simulink model "Spider_4leg_rotate_Ver0"  (R2024a)
settings: Solver=ode4  StartTime=0.0  StopTime=path_duration  FixedStep=0.01  RelTol=1e-3
PostLoadFcn:
  | addpath(fileparts(get_param('Spider_4leg_rotate_Ver0','FileName')));
InitFcn:
  | % Record inline model settings for the viewer; algorithms do not read this struct.
  | v0Model = 'Spider_4leg_rotate_Ver0';
  | v0Rt = sfroot;
  | v0W = v0Rt.find('-isa','Stateflow.EMChart','Path',[v0Model '/WPG']);
  | v0I = v0Rt.find('-isa','Stateflow.EMChart','Path',[v0Model '/IK_spider']);
  | v0F = v0Rt.find('-isa','Stateflow.EMChart','Path',[v0Model '/FK_spider']);
  | v0C = v0Rt.find('-isa','Stateflow.EMChart','Path',[v0Model '/COM_spider']);
  | v0Read = @(s,n) str2double(regexp(s,['(?m)^\s*' n '\s*=\s*([-+0-9.eE]+)\s*;'],'tokens','once'));
  | % Parse only numeric vector literals; no code is evaluated.
  | v0Literal = regexp(v0W.Script,'(?m)^\s*phi_leg\s*=\s*\[([0-9.,\s]+)\]','tokens','once');
  | v0Phase = sscanf(strrep(v0Literal{1},',',' '),'%f')';
  | v0Literal = regexp(v0C.Script,'(?m)^\s*com_offset\s*=\s*\[([-+0-9.eE,\s]+)\]','tokens','once');
  | v0Offset = sscanf(strrep(v0Literal{1},',',' '),'%f')';
  | v0P = struct;
  | v0P.FORMAT_VERSION = 1;
  | v0P.L = [v0Read(v0I.Script,'l1'),v0Read(v0I.Script,'l2'),v0Read(v0I.Script,'l3')];
  | v0cd = v0Read(v0W.Script,'cd');
  | v0cr = v0Read(v0W.Script,'cr');
  | v0P.HIP = [v0cd/2 v0cr/2;v0cd/2 -v0cr/2;-v0cd/2 -v0cr/2;-v0cd/2 v0cr/2];
  | v0P.STANCE = [v0Read(v0W.Script,'dx0'),v0Read(v0W.Script,'dy0')];
  | v0Switch = get_param([v0Model '/Direction'],'sw');
  | assert(ismember(v0Switch,{'0','1'}),'Ver0: invalid turn switch.');
  | v0Direction = 2*str2double(v0Switch)-1;
  | v0Base = sscanf(regexprep(get_param([v0Model '/COM0'],'Value'),'[\[\],]',' '),'%f');
  | assert(numel(v0Base)==3,'Ver0: COM0 must be a numeric [X Y Z] vector.');
  | v0P.BODY_H = v0Base(3);
  | v0P.STEP = 0;
  | v0P.T = str2double(get_param([v0Model '/T'],'Value'));
  | v0P.V = 0;
  | v0P.LIFT = v0Read(v0W.Script,'h');
  | v0P.SHIFT_X = v0Read(v0W.Script,'L_shift');
  | v0P.SHIFT_Y = v0Read(v0W.Script,'W_shift');
  | v0P.PHI = v0Phase;
  | if v0Direction > 0
  |     v0P.PHI = v0Phase([2 1 4 3]);
  | end
  | v0P.PREP = v0Read(v0W.Script,'beta_prep');
  | v0P.SWING = v0Read(v0W.Script,'beta_swing');
  | v0P.TOUCH = v0Read(v0W.Script,'beta_touch');
  | v0P.HEADING_DEG = str2double(get_param([v0Model '/phi0'],'Value'));
  | v0P.DT = str2double(get_param(v0Model,'FixedStep'));
  | v0Angle = str2double(get_param([v0Model '/Angle'],'Value'));
  | v0N = str2double(get_param([v0Model '/N'],'Value'));
  | assert(isfinite(v0Angle) && v0Angle>0 && v0Angle<=90,'Ver0: Angle must be in (0,90] degrees.');
  | assert(isfinite(v0N) && v0N>=4 && v0N<=200 && v0N==floor(v0N),'Ver0: N must be an integer in [4,200].');
  | v0Period = v0N*v0P.T;
  | assignin(get_param(v0Model,'ModelWorkspace'),'path_duration',v0Period);
  | assignin(get_param(v0Model,'ModelWorkspace'),'path_record',[3 v0Angle*pi/180 0 v0Period v0Direction 1]);
  | v0Stop = get_param(v0Model,'StopTime');
  | if strcmp(v0Stop,'path_duration')
  |     v0StopValue = v0Period;
  | else
  |     v0StopValue = str2double(v0Stop);
  | end
  | assert(isfinite(v0StopValue) && v0StopValue>0,'Ver0: Stop Time must be path_duration or a positive number.');
  | v0P.N_CYCLES = (v0StopValue-str2double(get_param(v0Model,'StartTime')))/v0P.T;
  | v0P.MASS_BODY = v0Read(v0C.Script,'m0')/1000;
  | v0P.MASS_LINK = [v0Read(v0C.Script,'m1'),v0Read(v0C.Script,'m2'),v0Read(v0C.Script,'m3')]/1000;
  | v0P.COM_OFFSET = v0Offset;
  | v0P.MARGIN_GUIDE = 0.005;
  | v0P.JOINT_TRIM = [0 -7 6;0 1.5 -3;4 -8 8;-6 -6 5];
  | v0P.SERVO_LO = [20 30 30];
  | v0P.SERVO_HI = [165 150 150];
  | assert(v0cd==v0Read(v0F.Script,'cd') && v0cr==v0Read(v0F.Script,'cr'),'Ver0: body dimensions differ between WPG and FK.');
  | assert(isequal(v0P.L,[v0Read(v0F.Script,'l1'),v0Read(v0F.Script,'l2'),v0Read(v0F.Script,'l3')]),'Ver0: link lengths differ between IK and FK.');
  | assert(v0P.DT==v0Read(v0C.Script,'dt') && v0P.DT==str2double(get_param([v0Model '/Delay1'],'SampleTime')),'Ver0: time step differs between solver, COM and Delay1.');
  | assert(v0P.PREP==0.75 && isequal(v0P.PHI,[.75 .5 .25 0] + (v0Direction>0)*[-.25 .25 -.25 .25]) && v0P.PREP<v0P.SWING && v0P.SWING<v0P.TOUCH && v0P.TOUCH<1,'Ver0: invalid phase schedule.');
  | assert(isfinite(v0P.T) && v0P.T>0 && v0P.V==0 && v0P.DT>0 && all(isfinite(v0P.L)) && all(v0P.L>0),'Ver0: invalid numeric parameter.');
  | assignin(get_param(v0Model,'ModelWorkspace'),'P',v0P);
  | clear v0Model v0Rt v0W v0I v0F v0C v0Read v0Vector v0Literal v0Phase v0Offset v0P v0cd v0cr v0Base
  | v0Root = sfroot;
  | v0Ref = v0Root.find('-isa','Stateflow.EMChart','Path',['Spider_4leg_rotate_Ver0' '/COM_ref']);
  | v0Wpg = v0Root.find('-isa','Stateflow.EMChart','Path',['Spider_4leg_rotate_Ver0' '/WPG']);
  | v0A = extractAfter(string(v0Ref.Script),'function pose = path_pose');
  | v0B = extractAfter(string(v0Wpg.Script),'function pose = path_pose');
  | assert(v0A==v0B,'Ver0: path_pose differs between COM_ref and WPG.');
  | clear v0R v0U v0Length v0Type v0Period v0Stop v0StopValue v0Root v0Ref v0Wpg v0A v0B
  | 
  | clear v0Switch v0Direction
  | clear v0Angle v0N
model workspace (MAT data in the model file):
  P.FORMAT_VERSION = 1
  P.L = [0.039 0.072 0.108]
  P.HIP = [0.0465  0.0445; 0.0465  -0.0445; -0.0465  -0.0445; -0.0465  0.0445]
  P.STANCE = [0.053 0.053]
  P.BODY_H = 0.088
  P.STEP = 0
  P.T = 12
  P.V = 0
  P.LIFT = 0.03
  P.SHIFT_X = 0.008
  P.SHIFT_Y = 0.017
  P.PHI = [0.75 0.5 0.25 0]
  P.PREP = 0.75
  P.SWING = 0.8
  P.TOUCH = 0.92
  P.HEADING_DEG = 0
  P.DT = 0.01
  P.N_CYCLES = 10
  P.MASS_BODY = 0.2
  P.MASS_LINK = [0.0134 0.0134 0.0134]
  P.COM_OFFSET = [0 0 0]
  P.MARGIN_GUIDE = 0.005
  P.JOINT_TRIM = [0  -7  6; 0  1.5  -3; 4  -8  8; -6  -6  5]
  P.SERVO_LO = [20 30 30]
  P.SERVO_HI = [165 150 150]
  path_duration = 120
  path_record = [3 1.57079632679 0 120 1 1]
settings Model: Creator=Huan  LastModifiedBy=hamin
settings RTWCC: GPUComputeCapability=3.5

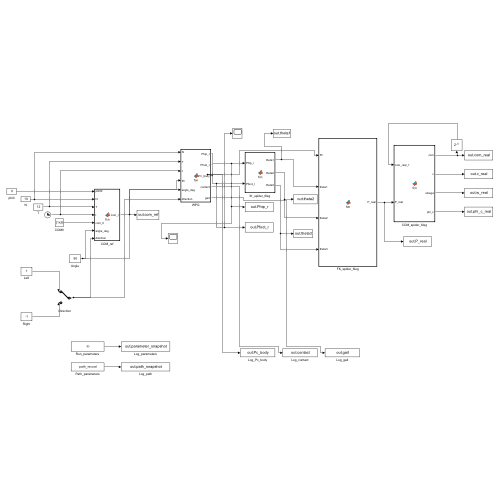
[thumbnail: Simulink's stored preview of the top-level diagram]
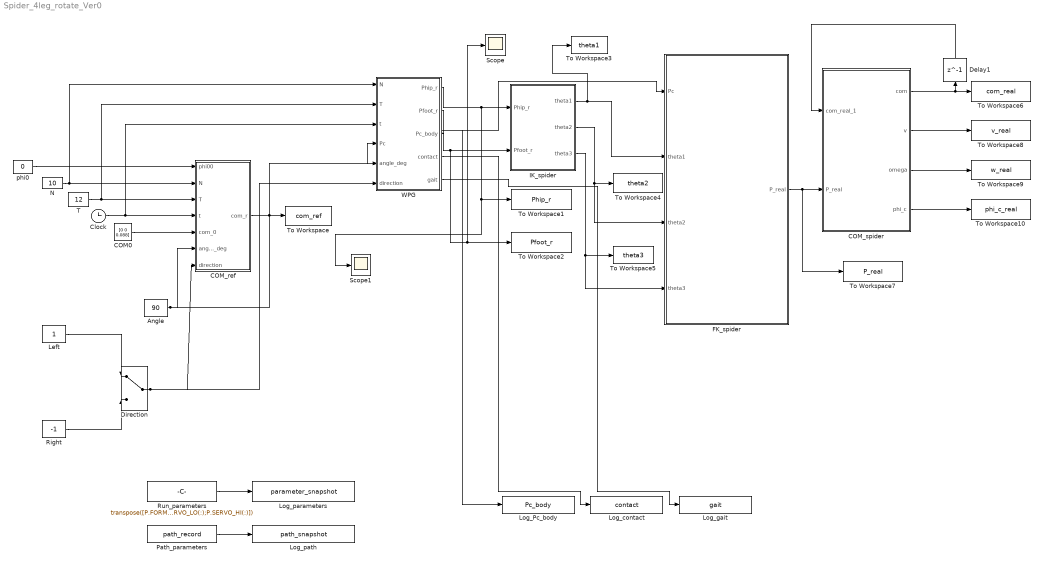
== system Spider_4leg_rotate_Ver0 ==
  Angle : Constant  Value=90
  COM0 : Constant  Value=[0 0 0.088]
  COM_ref : MATLAB Function  TreatAsAtomicUnit=on
  COM_spider : MATLAB Function  TreatAsAtomicUnit=on
  Clock : Clock
  Delay1 : Delay  DelayLength=1  InitialCondition=[0 0 -1 0]  SampleTime=0.01
  Direction : ManualSwitch
  FK_spider : MATLAB Function  TreatAsAtomicUnit=on
  IK_spider : MATLAB Function  TreatAsAtomicUnit=on
  Left : Constant
  Log_Pc_body : ToWorkspace  VariableName=Pc_body  SaveFormat=Timeseries  SampleTime=-1
  Log_contact : ToWorkspace  VariableName=contact  SaveFormat=Timeseries  SampleTime=-1
  Log_gait : ToWorkspace  VariableName=gait  SaveFormat=Timeseries  SampleTime=-1
  Log_parameters : ToWorkspace  VariableName=parameter_snapshot  SaveFormat=Timeseries  SampleTime=-1
      settings: MaxDataPoints=1
  Log_path : ToWorkspace  VariableName=path_snapshot  SaveFormat=Timeseries  SampleTime=-1
  N : Constant  Value=10
  Path_parameters : Constant  Value=path_record
  Right : Constant  Value=-1
  Run_parameters : Constant  Value=transpose([P.FORMAT_VERSION(:);P.L(:);P.HIP(:);P.STANCE(:);P.BODY_H(:);P.STEP(:);P.T(:);P.V(:);P.LIFT(:);P.SHIFT_X(:);P.SHIFT_Y(:);P.PHI(:);P.PREP(:);P.SWING(:);P.TOUCH(:);P.HEADING_DEG(:);P.DT(:);P.N_CYCLES(:);P.MASS_BODY(:);P.MASS_LINK(:);P.COM_OFFSET(:);P.MARGIN_GUIDE(:);P.JOINT_TRIM(:);P.SERVO_LO(:);P.SERVO_HI(:)])
  Scope : Scope
  Scope1 : Scope
  T : Constant  Value=12
  To Workspace : ToWorkspace  VariableName=com_ref  SaveFormat=Timeseries  SampleTime=-1
  To Workspace1 : ToWorkspace  VariableName=Phip_r  SaveFormat=Timeseries  SampleTime=-1
  To Workspace10 : ToWorkspace  VariableName=phi_c_real  SaveFormat=Timeseries  SampleTime=-1
  To Workspace2 : ToWorkspace  VariableName=Pfoot_r  SaveFormat=Timeseries  SampleTime=-1
  To Workspace3 : ToWorkspace  VariableName=theta1  SaveFormat=Timeseries  SampleTime=-1
  To Workspace4 : ToWorkspace  VariableName=theta2  SaveFormat=Timeseries  SampleTime=-1
  To Workspace5 : ToWorkspace  VariableName=theta3  SaveFormat=Timeseries  SampleTime=-1
  To Workspace6 : ToWorkspace  VariableName=com_real  SaveFormat=Timeseries  SampleTime=-1
  To Workspace7 : ToWorkspace  VariableName=P_real  SaveFormat=Timeseries  SampleTime=-1
  To Workspace8 : ToWorkspace  VariableName=v_real  SaveFormat=Timeseries  SampleTime=-1
  To Workspace9 : ToWorkspace  VariableName=w_real  SaveFormat=Timeseries  SampleTime=-1
  WPG : MATLAB Function  TreatAsAtomicUnit=on
  phi0 : Constant  Value=0
  wires:
  phi0/1 -> COM_ref/1(phi00)
  N/1 -> COM_ref/2(N), WPG/1(N)
  T/1 -> COM_ref/3(T), WPG/2(T)
  Clock/1 -> COM_ref/4(t), WPG/3(t)
  COM0/1 -> COM_ref/5(com_0)
  WPG/1(Phip_r) -> Scope1/1, To Workspace1/1, IK_spider/1(Phip_r)
  WPG/2(Pfoot_r) -> Scope/1, To Workspace2/1, IK_spider/2(Pfoot_r)
  IK_spider/1(theta1) -> To Workspace3/1, FK_spider/2(theta1)
  IK_spider/3(theta3) -> To Workspace5/1, FK_spider/4(theta3)
  Delay1/1 -> COM_spider/1(com_real_1)
  FK_spider/1(P_real) -> To Workspace7/1, COM_spider/2(P_real)
  COM_spider/1(com) -> To Workspace6/1, Delay1/1
  COM_ref/1(com_r) -> To Workspace/1, WPG/4(Pc)
  COM_spider/2(v) -> To Workspace8/1
  COM_spider/3(omega) -> To Workspace9/1
  COM_spider/4(phi_c) -> To Workspace10/1
  WPG/3(Pc_body) -> FK_spider/1(Pc), Log_Pc_body/1
  WPG/4(contact) -> Log_contact/1
  WPG/5(gait) -> Log_gait/1
  Run_parameters/1 -> Log_parameters/1
  IK_spider/2(theta2) -> FK_spider/3(theta2), To Workspace4/1
  Angle/1 -> WPG/5(angle_deg), COM_ref/6(angle_deg)
  Path_parameters/1 -> Log_path/1
  Left/1 -> Direction/1
  Right/1 -> Direction/2
  Direction/1 -> WPG/6(direction), COM_ref/7(direction)

== matlab function Spider_4leg_rotate_Ver0/IK_spider ==
  data: Phip_r input; theta1 output; Pfoot_r input; theta2 output; theta3 output
function [theta1, theta2, theta3] = fcn(Phip_r, Pfoot_r)
%% LEG LENGTH
l1 = 0.039;                    % Chieu dai khau 1 (m)
l2 = 0.072;                    % Chieu dai khau 2 (m)
l3 = 0.106;                    % Chieu dai khau 3 (m)
l = [l1, l2, l3];

%% INVERSE KINEMATICS OF FOUR LEGS
deta_leg1 = IK_spider(Phip_r(1,:), Pfoot_r(1,:), l);
deta_leg2 = IK_spider(Phip_r(2,:), Pfoot_r(2,:), l);
deta_leg3 = IK_spider(Phip_r(3,:), Pfoot_r(3,:), l);
deta_leg4 = IK_spider(Phip_r(4,:), Pfoot_r(4,:), l);

%% JOINT ANGLE OUTPUTS: 1 FL, 2 FR, 3 RR, 4 RL
theta1 = [deta_leg1(1), deta_leg2(1), deta_leg3(1), deta_leg4(1)];
theta2 = [deta_leg1(2), deta_leg2(2), deta_leg3(2), deta_leg4(2)];
theta3 = [deta_leg1(3), deta_leg2(3), deta_leg3(3), deta_leg4(3)];
end

function deta = IK_spider(Phip, Pfoot, l)
%% LOCAL FUNCTION: TOAN BO CONG THUC NAM TRONG KHOI NAY
% theta1 la phuong vi the gioi; theta3 chon nhanh goi am.
d = Pfoot(1:3) - Phip(1:3);
r = hypot(d(1), d(2));
a = d(3);
b = r - l(1);
c3 = (a*a + b*b - l(2)^2 - l(3)^2)/(2*l(2)*l(3));
assert(all(isfinite(d)) && r > l(1) && c3 >= -1-1e-10 && c3 <= 1+1e-10, ...
       'Ver0: IK target outside workspace.');
c3 = max(-1, min(1, c3));       % Chi chan sai so so hoc sat bien.
theta3 = atan2(-sqrt(max(0, 1-c3*c3)), c3);
theta2 = atan2(a, b) - atan2(l(3)*sin(theta3), l(2)+l(3)*cos(theta3));
theta1 = atan2(d(2), d(1));
deta = [theta1, theta2, theta3];
end

== matlab function Spider_4leg_rotate_Ver0/COM_ref ==
  data: phi00 input; N input; T input; t input; com_0 input; com_r output; angle_deg input; direction input size=1
function com_r = fcn(phi00, N, T, t, com_0, angle_deg, direction)
pose = path_pose(N, T, angle_deg, t, direction);
com_r = [com_0(1), com_0(2), com_0(3), phi00*pi/180+pose(3)];
end

function pose = path_pose(N, T, angle_deg, t, direction)
L = N-1;
z = min(L, max(0, t/T-0.5));
if z <= 0
    progress = 0;
elseif z >= L
    progress = 1;
elseif z < 1
    progress = 0.5*(z-sin(pi*z)/pi)/(L-1);
elseif z <= L-1
    progress = (z-0.5)/(L-1);
else
    r = L-z;
    progress = 1-0.5*(r-sin(pi*r)/pi)/(L-1);
end
pose = [0, 0, direction*angle_deg*pi/180*progress];
end

== matlab function Spider_4leg_rotate_Ver0/WPG ==
  data: N input; T input; t input; Pc input; Phip_r output; Pfoot_r output; Pc_body output; contact output; gait output; angle_deg input size=1; direction input size=1
function [Phip_r, Pfoot_r, Pc_body, contact, gait] = fcn(N, T, t, Pc, angle_deg, direction)
t = min(max(t,0),N*T);
%% BODY SHAPE
cd = 0.093;                     % Khoang cach hong truoc/sau (m)
cr = 0.089;                     % Khoang cach hong trai/phai (m)
Rbody = sqrt((cd/2)^2 + (cr/2)^2);
phi00 = atan2(cd, cr);

%% FOOT NEUTRAL OFFSETS
dx0 = 0.053;                    % Do mo chan so voi hong theo X (m)
dy0 = 0.053;                    % Do mo chan so voi hong theo Y (m)
% Chieu dai khau duoc khai bao truc tiep trong khoi IK va FK.

%% GAIT PARAMETERS
h = 0.030;                      % Chieu cao nhac chan (m)
frac = @(x) x - floor(x);

% MOC PHA RIENG CUA MOI CHAN:
% 0.75 <= s < 0.80: Pre-shift, 4 chan tru, tang bu than tu 0 den 1.
% 0.80 <= s < 0.92: Swing, 3 chan tru, giu muc bu than bang 1.
% 0.92 <= s < 1.00: Post-return, da ha chan, tra bu than tu 1 ve 0.
% 0.00 <= s < 0.75: Chan nay tru trong cac slot cua chan khac.
beta_prep = 0.75;
beta_swing = 0.80;
beta_touch = 0.92;
phi_leg = [0.75, 0.50, 0.25, 0.00];  % 1 FL, 2 FR, 3 RR, 4 RL
% CW/Right: FL -> FR -> RR -> RL; CCW/Left: FR -> FL -> RL -> RR.
if direction > 0
    phi_leg = phi_leg([2 1 4 3]);  % Mirror the schedule, not leg identities.
end

%% ROTATION
yaw = Pc(4);
Rz = [cos(yaw), -sin(yaw);
      sin(yaw),  cos(yaw)];

%% LEG MOUNT ANGLES
phi = [phi00, pi - phi00, pi + phi00, 2*pi - phi00];

%% HIP POSITIONS BEFORE BODY SHIFT
Phip_r = zeros(4, 4);
for i = 1:4
    p_local = [Rbody * sin(phi(i)); Rbody * cos(phi(i))];
    p_rot = Rz * p_local;
    Phip_r(i, :) = [Pc(1) + p_rot(1), Pc(2) + p_rot(2), ...
                   Pc(3), atan2(p_local(2), p_local(1)) + yaw];
end

%% PHASE VALUES
% Lam tron sai so so hoc sat moc pha, tranh doi chan muon mot mau.
phase = zeros(1, 4);
edges = [0, beta_prep, beta_swing, beta_touch, 1];
for i = 1:4
    phase(i) = frac(t/T + phi_leg(i));
    for e = 1:5
        if abs(phase(i) - edges(e)) < 1e-12
            phase(i) = edges(e);
        end
    end
    if phase(i) == 1
        phase(i) = 0;
    end
end

%% XAC DINH TRANG THAI DOI THAN
x_shift_body = 0;
y_shift_body = 0;
W_shift = 0.017;                % Bien do bu ngang (m)
L_shift = 0.008;                % Bien do bu doc (m)
dir_x = [ 1,  1,-1,-1];
dir_y = [ 1, -1,-1, 1];
active_leg = 1;
stage = 1;

for k = 1:4
    s_k = phase(k);
    if (s_k >= beta_prep) && (s_k < 1.00)
        active_leg = k;
        if s_k < beta_swing
            % PHA 1: PRE-SHIFT, van toc bu bang 0 o hai dau.
            tau = (s_k - beta_prep)/(beta_swing - beta_prep);
            shift_val = 0.5 - 0.5*cos(pi*tau);
            stage = 1;
        elseif s_k < beta_touch
            % PHA 2: SWING, giu bu than.
            shift_val = 1.0;
            stage = 2;
        else
            % PHA 3: POST-RETURN, tra bu ve 0 mot cach lien tuc.
            tau = (s_k - beta_touch)/(1.00 - beta_touch);
            shift_val = 0.5 + 0.5*cos(pi*tau);
            stage = 3;
        end
        x_shift_body = dir_x(k)*L_shift*shift_val;
        y_shift_body = dir_y(k)*W_shift*shift_val;
        break;
    end
end

%% APPLY ONE BODY SHIFT TO ALL HIPS AND FK
% Bu chan +offset trong he than tuong duong than dich -offset tren mat dat.
% Khong cong offset vao diem chan da bam dat, ke ca chan sap nhac/vua ha.
shift_world = -Rz*[x_shift_body; y_shift_body];
Pc_body = [Pc(1) + shift_world(1), Pc(2) + shift_world(2), Pc(3), yaw];
for i = 1:4
    Phip_r(i, 1:2) = Phip_r(i, 1:2) + shift_world';
end

%% TINH QUY DAO TUNG CHAN
% Suy goc xoay va goc toa do tu tham chieu hien tai.
% Moi neo chan la mot diem THE GIOI, giu nguyen suot pha stance.
pose_now = path_pose(N, T, angle_deg, t, direction);
heading0 = yaw - pose_now(3);
R0 = [cos(heading0), -sin(heading0); sin(heading0), cos(heading0)];
origin = [Pc(1); Pc(2)] - R0*pose_now(1:2)';
Pfoot_r = zeros(4, 3);
contact = ones(1, 4);
swing_leg = 0;
T_stance = 1.0 - (beta_touch - beta_swing);

for i = 1:4
    s = phase(i);
    p_hip = [Rbody*sin(phi(i)); Rbody*cos(phi(i))];
    p_local = p_hip + [sign(p_hip(1))*dx0; sign(p_hip(2))*dy0];
    if (s >= beta_swing) && (s < beta_touch)
        % SWING: noi hai neo bang cycloid, van toc 0 khi nhac/ha.
        ss = (s-beta_swing)/(beta_touch-beta_swing);
        touchdown_t = t + (1-ss)*(beta_touch-beta_swing)*T;
        next_mid_t = touchdown_t + T_stance*T/2;
        a = foot_anchor(N, T, angle_deg, next_mid_t-T, p_local, direction);
        b = foot_anchor(N, T, angle_deg, next_mid_t, p_local, direction);
        progress = ss - sin(2*pi*ss)/(2*pi);
        xy = a + (b-a)*progress;
        zs = h*sin(pi*ss)^2;
        contact(i) = 0;
        swing_leg = i;
    else
        % STANCE: thoi diem giua stance khong doi trong ca khoang tru.
        if s >= beta_touch
            tau_st = s-beta_touch;
        else
            tau_st = (1-beta_touch)+s;
        end
        mid_t = t-tau_st*T+T_stance*T/2;
        xy = foot_anchor(N, T, angle_deg, mid_t, p_local, direction);
        zs = 0;
    end
    xy_world = origin + R0*xy;
    Pfoot_r(i,:) = [xy_world', zs];
end
gait = [active_leg, stage, swing_leg, -x_shift_body, -y_shift_body];
end

function xy = foot_anchor(N, T, angle_deg, mid_t, p_local, direction)
pose = path_pose(N, T, angle_deg, mid_t, direction);
R = [cos(pose(3)), -sin(pose(3)); sin(pose(3)), cos(pose(3))];
xy = pose(1:2)' + R*p_local;
end

function pose = path_pose(N, T, angle_deg, t, direction)
L = N-1;
z = min(L, max(0, t/T-0.5));
if z <= 0
    progress = 0;
elseif z >= L
    progress = 1;
elseif z < 1
    progress = 0.5*(z-sin(pi*z)/pi)/(L-1);
elseif z <= L-1
    progress = (z-0.5)/(L-1);
else
    r = L-z;
    progress = 1-0.5*(r-sin(pi*r)/pi)/(L-1);
end
pose = [0, 0, direction*angle_deg*pi/180*progress];
end

== matlab function Spider_4leg_rotate_Ver0/FK_spider ==
  data: Pc input; theta1 input; theta2 input; theta3 input; P_real output
function P_real = fcn(Pc, theta1, theta2, theta3)
%% BODY SHAPE
cd = 0.093;
cr = 0.089;
R_new = sqrt((cd/2)^2 + (cr/2)^2);
phi00 = atan2(cd, cr);

%% LEG LENGTH
l1 = 0.039;
l2 = 0.072;
l3 = 0.106;
l = [l1, l2, l3];

%% HIP POSITIONS
% Pc nhan truc tiep Pc_body cua WPG, da bao gom dich than.
phi = [phi00, pi - phi00, pi + phi00, 2*pi - phi00];
Rz = [cos(Pc(4)), -sin(Pc(4));
      sin(Pc(4)),  cos(Pc(4))];
Phip = zeros(4, 4);
for i = 1:4
    p_local = [R_new*sin(phi(i)); R_new*cos(phi(i))];
    p_rot = Rz*p_local;
    Phip(i,:) = [Pc(1)+p_rot(1), Pc(2)+p_rot(2), Pc(3), ...
                atan2(p_local(2), p_local(1))+Pc(4)];
end
P10 = Phip(1,:);
P20 = Phip(2,:);
P30 = Phip(3,:);
P40 = Phip(4,:);

%% FORWARD KINEMATICS OF FOUR LEGS
[P10, P11, P12, P13] = FK_spider(P10, l, [theta1(1), theta2(1), theta3(1)]);
[P20, P21, P22, P23] = FK_spider(P20, l, [theta1(2), theta2(2), theta3(2)]);
[P30, P31, P32, P33] = FK_spider(P30, l, [theta1(3), theta2(3), theta3(3)]);
[P40, P41, P42, P43] = FK_spider(P40, l, [theta1(4), theta2(4), theta3(4)]);
P_real = [P10, P11, P12, P13, P20, P21, P22, P23, ...
          P30, P31, P32, P33, P40, P41, P42, P43];
end

function [P0, P1, P2, P3] = FK_spider(P0, l, theta)
%% LOCAL FUNCTION: TOAN BO CONG THUC NAM TRONG KHOI NAY
theta1 = theta(1);
theta2 = theta(2);
theta3 = theta(3);
e = [cos(theta1), sin(theta1)];
% theta1 da la phuong vi the gioi, khong cong goc lap hong lan nua.
P1 = [P0(1:2)+l(1)*e, P0(3), theta1];
P2 = [P1(1:2)+l(2)*cos(theta2)*e, P1(3)+l(2)*sin(theta2), theta1];
P3 = [P2(1:2)+l(3)*cos(theta2+theta3)*e, ...
      P2(3)+l(3)*sin(theta2+theta3), theta1];
end

== matlab function Spider_4leg_rotate_Ver0/COM_spider ==
  data: com_real_1 input; P_real input; com output; v output; omega output; phi_c output
function [com,v,omega,phi_c]   = fcn(com_real_1,P_real)
%% MASS ASSUMPTIONS (g), CHUA CAN DO ROBOT THAT
m0 = 200;
m1 = 13.4;
m2 = 13.4;
m3 = 13.4;
M = [m1 m2 m3 m1 m2 m3 m1 m2 m3 m1 m2 m3 m0];

P1_leg1 = P_real(1:4);
P2_leg1 = P_real(5:8);
P3_leg1 = P_real(9:12);
P4_leg1 = P_real(13:16);

P1_leg2 = P_real(17:20);
P2_leg2 = P_real(21:24);
P3_leg2 = P_real(25:28);
P4_leg2 = P_real(29:32);

P1_leg3 = P_real(33:36);
P2_leg3 = P_real(37:40);
P3_leg3 = P_real(41:44);
P4_leg3 = P_real(45:48);

P1_leg4 = P_real(49:52);
P2_leg4 = P_real(53:56);
P3_leg4 = P_real(57:60);
P4_leg4 = P_real(61:64);

% tinh khoi tam
% chan 1
PP12_leg1.x = (P1_leg1(:,1) + P2_leg1(:,1))/2;
PP12_leg1.y = (P1_leg1(:,2) + P2_leg1(:,2))/2;
PP12_leg1.z = (P1_leg1(:,3) + P2_leg1(:,3))/2;

PP23_leg1.x = (P2_leg1(:,1) + P3_leg1(:,1))/2;
PP23_leg1.y = (P2_leg1(:,2) + P3_leg1(:,2))/2;
PP23_leg1.z = (P2_leg1(:,3) + P3_leg1(:,3))/2;

PP34_leg1.x = (P3_leg1(:,1) + P4_leg1(:,1))/2;
PP34_leg1.y = (P3_leg1(:,2) + P4_leg1(:,2))/2;
PP34_leg1.z = (P3_leg1(:,3) + P4_leg1(:,3))/2;

% chan 2
PP12_leg2.x = (P1_leg2(:,1) + P2_leg2(:,1))/2;
PP12_leg2.y = (P1_leg2(:,2) + P2_leg2(:,2))/2;
PP12_leg2.z = (P1_leg2(:,3) + P2_leg2(:,3))/2;

PP23_leg2.x = (P2_leg2(:,1) + P3_leg2(:,1))/2;
PP23_leg2.y = (P2_leg2(:,2) + P3_leg2(:,2))/2;
PP23_leg2.z = (P2_leg2(:,3) + P3_leg2(:,3))/2;

PP34_leg2.x = (P3_leg2(:,1) + P4_leg2(:,1))/2;
PP34_leg2.y = (P3_leg2(:,2) + P4_leg2(:,2))/2;
PP34_leg2.z = (P3_leg2(:,3) + P4_leg2(:,3))/2;

% chan 3
PP12_leg3.x = (P1_leg3(:,1) + P2_leg3(:,1))/2;
PP12_leg3.y = (P1_leg3(:,2) + P2_leg3(:,2))/2;
PP12_leg3.z = (P1_leg3(:,3) + P2_leg3(:,3))/2;

PP23_leg3.x = (P2_leg3(:,1) + P3_leg3(:,1))/2;
PP23_leg3.y = (P2_leg3(:,2) + P3_leg3(:,2))/2;
PP23_leg3.z = (P2_leg3(:,3) + P3_leg3(:,3))/2;

PP34_leg3.x = (P3_leg3(:,1) + P4_leg3(:,1))/2;
PP34_leg3.y = (P3_leg3(:,2) + P4_leg3(:,2))/2;
PP34_leg3.z = (P3_leg3(:,3) + P4_leg3(:,3))/2;

% chan 4
PP12_leg4.x = (P1_leg4(:,1) + P2_leg4(:,1))/2;
PP12_leg4.y = (P1_leg4(:,2) + P2_leg4(:,2))/2;
PP12_leg4.z = (P1_leg4(:,3) + P2_leg4(:,3))/2;

PP23_leg4.x = (P2_leg4(:,1) + P3_leg4(:,1))/2;
PP23_leg4.y = (P2_leg4(:,2) + P3_leg4(:,2))/2;
PP23_leg4.z = (P2_leg4(:,3) + P3_leg4(:,3))/2;

PP34_leg4.x = (P3_leg4(:,1) + P4_leg4(:,1))/2;
PP34_leg4.y = (P3_leg4(:,2) + P4_leg4(:,2))/2;
PP34_leg4.z = (P3_leg4(:,3) + P4_leg4(:,3))/2;

%% BODY CENTER AND OFFSET
com_offset = [0, 0, 0]; % (m), he than
phi_c = atan2(-(P1_leg1(1)-P1_leg2(1)), P1_leg1(2)-P1_leg2(2));
Rz = [cos(phi_c), -sin(phi_c); sin(phi_c), cos(phi_c)];
offset_xy = Rz*com_offset(1:2)';
% than
PPM.x=(P1_leg1(:,1)+ P1_leg2(:,1)+ P1_leg3(:,1)+ P1_leg4(:,1))/4;
PPM.y=(P1_leg1(:,2)+ P1_leg2(:,2)+ P1_leg3(:,2)+ P1_leg4(:,2))/4;
PPM.z=(P1_leg1(:,3)+ P1_leg2(:,3)+ P1_leg3(:,3)+ P1_leg4(:,3))/4;

PPM.x = PPM.x + offset_xy(1);
PPM.y = PPM.y + offset_xy(2);
PPM.z = PPM.z + com_offset(3);

PPx = [PP12_leg1.x PP23_leg1.x PP34_leg1.x PP12_leg2.x PP23_leg2.x PP34_leg2.x PP12_leg3.x PP23_leg3.x PP34_leg3.x PP12_leg4.x PP23_leg4.x PP34_leg4.x PPM.x];
PPy = [PP12_leg1.y PP23_leg1.y PP34_leg1.y PP12_leg2.y PP23_leg2.y PP34_leg2.y PP12_leg3.y PP23_leg3.y PP34_leg3.y PP12_leg4.y PP23_leg4.y PP34_leg4.y PPM.y];
PPz = [PP12_leg1.z PP23_leg1.z PP34_leg1.z PP12_leg2.z PP23_leg2.z PP34_leg2.z PP12_leg3.z PP23_leg3.z PP34_leg3.z PP12_leg4.z PP23_leg4.z PP34_leg4.z PPM.z];

comx_real = M*PPx'/sum(M);
comy_real = M*PPy'/sum(M);
comz_real = M*PPz'/sum(M);
%% VELOCITY AND HEADING
dt = 0.01;                      % Dong bo voi Fixed-step size va Delay1.
% Huong than lay tu hong; khong coi huong lac COM la yaw cua than.
if com_real_1(3) < 0
    v = 0;                       % Bo xung gia o mau dau.
    omega = 0;
else
    dx = comx_real - com_real_1(1);
    dy = comy_real - com_real_1(2);
    v = hypot(dx, dy)/dt;
    dphi = phi_c - com_real_1(4);
    omega = atan2(sin(dphi), cos(dphi))/dt;
end
com = [comx_real, comy_real, comz_real, phi_c];
end
